simulink model "basic_IO_qarm_mini"  (R2024a)
settings: Solver=ode1  StartTime=0.0  StopTime=inf  FixedStep=1/30  RelTol=1e-3  EnableMultiTasking=on
undefined symbols (not defined in the file): gcbh, HIL, JPEG, qc_get_step_size, video_display_show
libraries: quarc_library x11, simulink x1
settings Model: Creator=msaravanan  LastModifiedBy=Edu-Sivamani
settings SolverCC: PositivePriorityOrder=on
settings HardwareCC: ProdBitPerLong=64  ProdLargestAtomicInteger=LongLong  ProdLargestAtomicFloat=Double  ProdLongLongMode=on  ProdHWDeviceType=ARM Compatible->ARM 64-bit (LP64)
settings RTWCC: Description=QUARC Linux QBot Platform Target Using Toolchain  SystemTargetFile=quarc_linux_qbot_platform.tlc  Toolchain=QUARC linux_qbot_platform | gmake (64-bit Windows)  BuildConfiguration=Faster Runs
settings STFCustomTargetCC: ConcurrentExecutionCompliant=on  SystemTargetFile=quarc_linux_qbot_platform.tlc
settings GRTTargetCC: ParMdlRefBuildCompliant=off  CompOptLevelCompliant=off  CombineOutputUpdateFcns=off  MatFileLogging=off  CPPClassGenCompliant=off  GRTInterface=on  ExtMode=on  ExtModeMexFile=quarc_comm  ExtModeMexArgs='-w -d /tmp -uri %u','tcpip://192.168.2.101:17002'

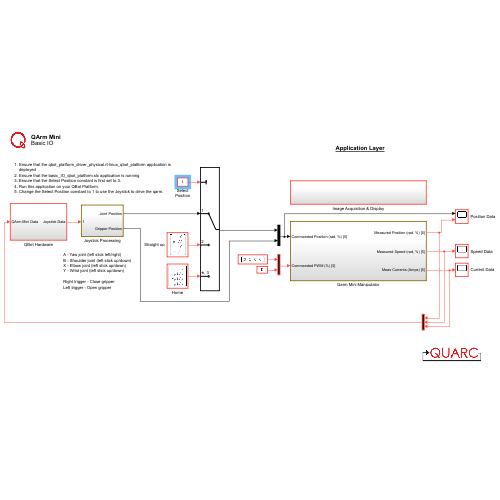
[thumbnail: Simulink's stored preview of the top-level diagram]
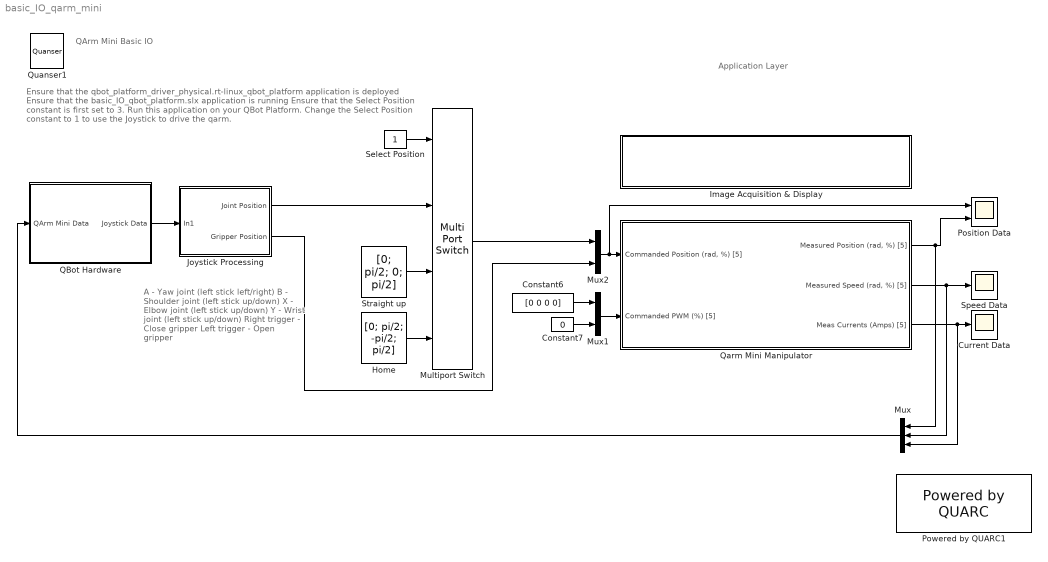
== system basic_IO_qarm_mini ==
  note: A - Yaw joint (left stick left/right)
      | B - Shoulder joint (left stick up/down)
      | X - Elbow joint (left stick up/down)
      | Y - Wrist joint (left stick up/down)
      |
      | Right trigger - Close gripper
      | Left trigger - Open gripper
  note: Ensure that the qbot_platform_driver_physical.rt-linux_qbot_platform application is deployed
      | Ensure that the basic_IO_qbot_platform.slx application is running
      | Ensure that the Select Position constant is first set to 3.
      | Run this application on your QBot Platform.
      | Change the Select Position constant to 1 to use the Joystick to drive the qarm.
  note: QArm Mini
      | Basic IO
  note: Application Layer
  Constant6 : Constant  Value=[0 0 0 0]  SampleTime=qc_get_step_size
  Constant7 : Constant  Value=0  SampleTime=qc_get_step_size
  Current Data : Scope
  Home : Constant  Value=[0; pi/2; -pi/2; pi/2]  VectorParams1D=off  SampleTime=qc_get_step_size
  Image Acquisition & Display : Subsystem
  Joystick Processing : Subsystem
  Multiport Switch : MultiPortSwitch  SaturateOnIntegerOverflow=off  InputSameDT=off
  Mux : Mux  Inputs=3
  Mux1 : Mux  Inputs=2
  Mux2 : Mux  Inputs=2
  Position Data : Scope  NumInputPorts=2
  Powered by QUARC1 : quarc_library/Logos/Powered by QUARC
  QBot Hardware : Subsystem
  Qarm Mini Manipulator : Subsystem
  Quanser1 : quarc_library/Logos/Quanser
  Select Position : Constant  SampleTime=qc_get_step_size
  Speed Data : Scope
  Straight up : Constant  Value=[0; pi/2; 0; pi/2]  VectorParams1D=off  SampleTime=qc_get_step_size
  wires:
  Mux2/1 -> Position Data/1, Qarm Mini Manipulator/1("Commanded Position (rad, %) [5]")
  Constant7/1 -> Mux1/2
  Joystick Processing/2(Gripper Position) -> Mux2/2
  Mux1/1 -> Qarm Mini Manipulator/2(Commanded PWM (%) [5])
  Constant6/1 -> Mux1/1
  Multiport Switch/1 -> Mux2/1
  Qarm Mini Manipulator/1("Measured Position (rad, %) [5]") -> Mux/1, Position Data/2
  Qarm Mini Manipulator/3(Meas Currents (Amps) [5]) -> Mux/3, Current Data/1
  Qarm Mini Manipulator/2("Measured Speed (rad, %) [5]") -> Mux/2, Speed Data/1
  Straight up/1 -> Multiport Switch/3
  QBot Hardware/1(Joystick Data) -> Joystick Processing/1(In1)
  Select Position/1 -> Multiport Switch/1
  Home/1 -> Multiport Switch/4
  Joystick Processing/1(Joint Position) -> Multiport Switch/2
  Mux/1 -> QBot Hardware/1(QArm Mini Data)

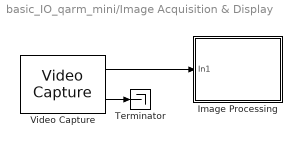
== system basic_IO_qarm_mini/Image Acquisition & Display ==
  Image Processing : Subsystem  LoadFcn=set_param(gcbh, 'UserData', gcb);  StartFcn=video_display_show([gcb, '/Video Display'], 'add', gcb);  mask(Video Compressed Display){algorithm=JPEG, quality=50, sample_time=-1, use_hardware=on}
      mask prompts: algorithm "Compression algorithm:"; quality "Compression quality (0-100):"; sample_time "Sample time (seconds):"; use_hardware "Use hardware acceleration for video display"
      mask help: Displays a video stream on the host, using compression to minimize bandwidth.
      mask init:
      | qc_set_display('Video\nCompressed\nDisplay');
      settings: UndoDeleteFcn=set_param(gcbh, 'UserData', gcb);  OpenFcn=video_display_show([gcb, '/Video Display'], 'show', gcb);  PreDeleteFcn=video_display_show([gcb, '/Video Display'], 'delete');
      settings: CopyFcn=|
      | set_param(gcbh, 'UserData', gcb);
      | set_param(gcbh, 'LinkStatus', 'none');
      settings: NameChangeFcn=|
      | video_display_show([get_param(gcbh, 'UserData'), '/Video Display'], 'rename', [gcb, '/Video Display']);
      | video_display_show([gcb, '/Video Display'], 'add', gcb);
      | set_param(gcbh, 'UserData', gcb);
      mask Help: web(qc_get_block_help_path(gcb));
      mask TypeOptions algorithm: Image Compress/algorithm
      mask TypeOptions quality: Image Compress/quality
      mask TypeOptions sample_time: Video Display/sample_time
      mask TypeOptions use_hardware: Video Display/use_hardware
      mask Display:
      | patch([0.98591 0.98591 0.62618 0.59072 0.56147   0.536   0.536  0.5441 0.56912 0.59207 0.60881 0.62276 0.63527 0.64364  0.6485  0.6485 0.64706 0.64499 0.63662 0.62411 0.61232 0.59837 0.58307 0.56147   0.536   0.536  0.5441  0.5747 0.60953 0.63662 0.67001  0.7034 0.72851 0.75425 0.77927 0.80294 0.82454 0.84119 0.85865 0.87395 0.88574 0.89339  0.8969 0.89969 0.89969 0.89267  0.8816 0.87044 0.85649  0.8384 0.81824 0.80294 0.78764 0.77513 0.76676 0.75776 0.76397 0.77513 0.79178 0.80987 0.82796 0.84326 0.86207 0.98528],[0.18689 0.05522 0.05522 0.05171 0.05171    0.05 0.18338 0.18338 0.19148 0.20435 0.22298 0.24863 0.28589 0.33125 0.38138 0.55139 0.59801 0.63761 0.68189 0.72149 0.74939 0.76694 0.77855 0.79367 0.79952 0.92768 0.92768 0.92768 0.92417 0.92066 0.91364  0.9032 0.89384 0.88106 0.86594 0.85073 0.82634 0.80537 0.77855 0.74363 0.70403 0.65858 0.61079 0.59099 0.41513 0.37202 0.31847 0.29048 0.25556 0.23342  0.2102 0.19382 0.18221 0.17285 0.16943 0.16124  0.1589 0.16241 0.16709 0.17168  0.1787 0.18221 0.18689 0.18689],[0.9,0.90,0.91])
      | patch([0.536 0.52601 0.46823 0.44528 0.41603 0.39101 0.35555 0.33116 0.31451 0.29291  0.2804 0.26717 0.25322 0.23999 0.22406 0.20732 0.19337 0.17528 0.15935 0.14396 0.13217 0.11759 0.10922 0.10085 0.09671 0.09392 0.09041 0.08906 0.08906 0.09464  0.0995 0.10778 0.11894 0.13145 0.14675 0.16349 0.17672 0.19409 0.20732 0.22406 0.23999 0.26159 0.27833 0.29849 0.31793 0.33602 0.35411 0.37085 0.39245 0.41603   0.536   0.536 0.53159 0.46409   0.446 0.42026 0.39587 0.37571 0.36113 0.34925 0.34088 0.33809 0.33809 0.34088 0.34583 0.35627 0.36392 0.38129 0.39587 0.41117 0.42719 0.44672  0.4676 0.48353 0.48353 0.52394   0.536],[0.05 0.04829 0.04712 0.04712 0.04829 0.05063 0.05405 0.05873 0.06107 0.06692 0.07043 0.07619 0.08087 0.08672 0.09482 0.10652 0.11696 0.13325  0.1508 0.17168 0.19499 0.22415 0.25439 0.28472 0.31379 0.35456 0.38489 0.41513 0.58055 0.63878 0.68774 0.72149 0.75641 0.78089 0.80537 0.82859 0.84029 0.85658 0.86594 0.87404  0.8834 0.89267 0.90086 0.90788 0.91247 0.91832 0.92066   0.923 0.92651 0.92768 0.92768 0.79952 0.79952 0.79952 0.79718 0.78899 0.77153 0.75056 0.72149 0.68072 0.62249  0.5549 0.41396 0.37085 0.33242 0.28121 0.25205 0.22181 0.20552 0.19499 0.18572 0.18221 0.17753 0.17636 0.17753  0.1787  0.1787],[0.9,0.90,0.91])
      | disp('Video\nCompressed\nDisplay');
  Terminator : Terminator
  Video Capture : quarc_library/Multimedia/Video Capture  source=device  device=7  filename=sample_movie.mov  value=[0 0; 0 0]  resolution=640 x 360  width=640  height=360  output_format=MATLAB RGB (HxWx3)  data_type=uint8  sample_time=qc_get_step_size * ceil(1 / 60.0 / qc_get_step_size)  brightness_override=Do not override  brightness=50.0  contrast_override=Do not override  contrast=50.0  hue_override=Do not override  hue=50.0  saturation_override=Do not override  saturation=50.0  sharpness_override=Do not override  sharpness=50.0  gamma_override=Do not override  gamma=50.0  coloreffect_override=Do not override  coloreffect=None  whitebalance_override=Do not override  whitebalance=50.0  backlightcompensation_override=Do not override  backlightcompensation=0.0  gain_override=Do not override  gain=50.0  pan_override=Do not override  pan=50.0  tilt_override=Do not override  tilt=50.0  roll_override=Do not override  roll=50.0  zoom_override=Do not override  zoom=0.0  exposure_override=Do not override  exposure=50.0  iris_override=Do not override  iris=50.0  mirror_override=Do not override  mirror=None  focus_override=Do not override  focus=0.0
      settings: SourceProductName=QUARC Targets
  wires:
  Video Capture/1 -> Image Processing/1(In1)
  Video Capture/2 -> Terminator/1

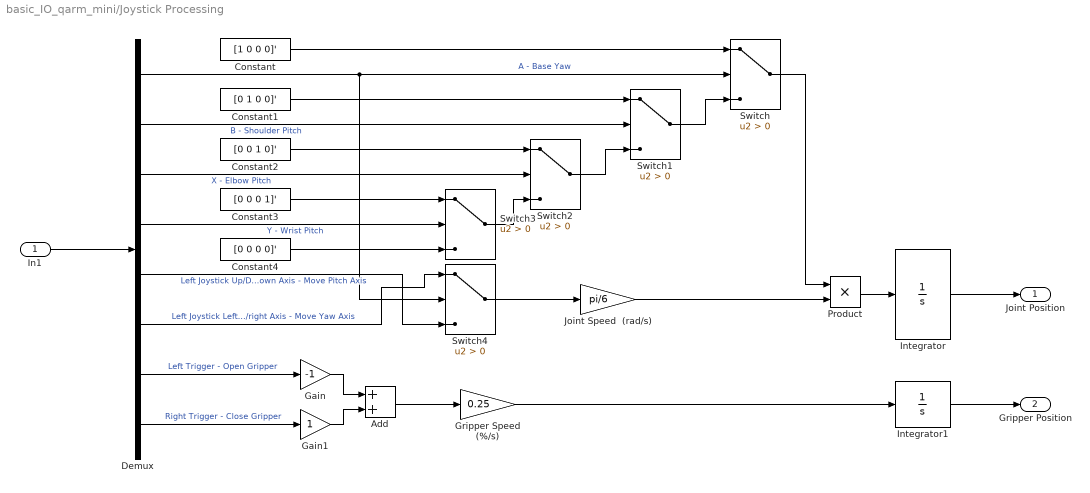
== system basic_IO_qarm_mini/Joystick Processing ==
  In1 : Inport
  Add : Sum
  Constant : Constant  Value=[1 0 0 0]'
  Constant1 : Constant  Value=[0 1 0 0]'
  Constant2 : Constant  Value=[0 0 1 0]'
  Constant3 : Constant  Value=[0 0 0 1]'
  Constant4 : Constant  Value=[0 0 0 0]'
  Demux : Demux  Outputs=8
  Gain : Gain  Gain=-1
  Gain1 : Gain
  Gripper Speed (%/s) : Gain  Gain=0.25
  Integrator : Integrator  InitialCondition=[0; pi/2; -pi/2; pi/2]  LimitOutput=on  UpperSaturationLimit=[5*pi/4, pi, 0, 3*pi/4]'  LowerSaturationLimit=[-pi/2. 0, -3*pi/4, 0]'
  Integrator1 : Integrator  InitialCondition=0.5  LimitOutput=on  UpperSaturationLimit=1  LowerSaturationLimit=0
  Joint Speed  (rad/s) : Gain  Gain=pi/6
  Product : Product
  Switch{,1..4} (5 alike) : Switch  Criteria=u2 > Threshold  SaturateOnIntegerOverflow=off  InputSameDT=off
  Joint Position : Outport
  Gripper Position : Outport  Port=2
  wires:
  In1/1 -> Demux/1
  Demux/1 -> Switch4/2, Switch/2  "A - Base Yaw"
  Constant/1 -> Switch/1
  Switch1/1 -> Switch/3
  Demux/2 -> Switch1/2  "B - Shoulder Pitch"
  Constant1/1 -> Switch1/1
  Demux/3 -> Switch2/2  "X - Elbow Pitch"
  Demux/4 -> Switch3/2  "Y - Wrist Pitch"
  Constant2/1 -> Switch2/1
  Constant3/1 -> Switch3/1
  Constant4/1 -> Switch3/3
  Demux/5 -> Switch4/3  "Left Joystick Up/Down Axis - Move Pitch Axis"
  Demux/6 -> Switch4/1  "Left Joystick Left/right Axis - Move Yaw Axis"
  Switch2/1 -> Switch1/3
  Switch3/1 -> Switch2/3
  Switch4/1 -> Joint Speed  (rad/s)/1
  Switch/1 -> Product/1
  Joint Speed  (rad/s)/1 -> Product/2
  Product/1 -> Integrator/1
  Integrator/1 -> Joint Position/1
  Demux/7 -> Gain/1  "Left Trigger - Open Gripper"
  Demux/8 -> Gain1/1  "Right Trigger - Close Gripper"
  Gain/1 -> Add/1
  Gain1/1 -> Add/2
  Add/1 -> Gripper Speed (%/s)/1
  Gripper Speed (%/s)/1 -> Integrator1/1
  Integrator1/1 -> Gripper Position/1

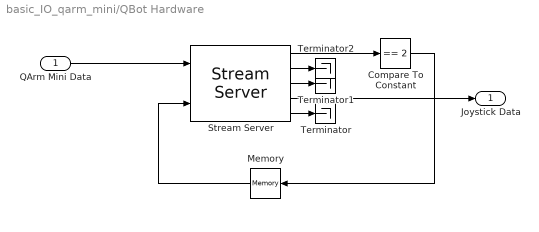
== system basic_IO_qarm_mini/QBot Hardware ==
  QArm Mini Data : Inport
  Compare To Constant : simulink/Logic and Bit Operations/Compare To Constant  relop===  const=2  OutDataTypeStr=boolean
  Memory : Memory  InheritSampleTime=on
  Stream Server : quarc_library/Communications/Basic/Stream Server  uri_source=Specify via dialog (do not evaluate)  uri=tcpip://localhost:18889  send_buffer_size=15*8  receive_buffer_size=8*8  byte_order=little endian (Intel - LSB first)  optimization=Minimum latency  send_options=Send most recent data  receive_options=Receive most recent data  default_value=zeros(1,8)  sample_time=qc_get_step_size  active=on  implementation=Use blocking I/O in a separate thread  send_fifo_size=1000  receive_fifo_size=1000  send_priority=0  receive_priority=0  send_dimensions=off  receive_dimensions=off  max_dimensions=-1  data_type=Inherited via back propagation  type_expr=BusObject
      settings: AttributesFormatString="\"tcpip://localhost:18889\""
  Terminator : Terminator
  Terminator1 : Terminator
  Terminator2 : Terminator
  Joystick Data : Outport
  wires:
  Stream Server/1 -> Compare To Constant/1
  QArm Mini Data/1 -> Stream Server/1
  Compare To Constant/1 -> Memory/1
  Memory/1 -> Stream Server/2
  Stream Server/4 -> Joystick Data/1
  Stream Server/5 -> Terminator/1
  Stream Server/3 -> Terminator1/1
  Stream Server/2 -> Terminator2/1

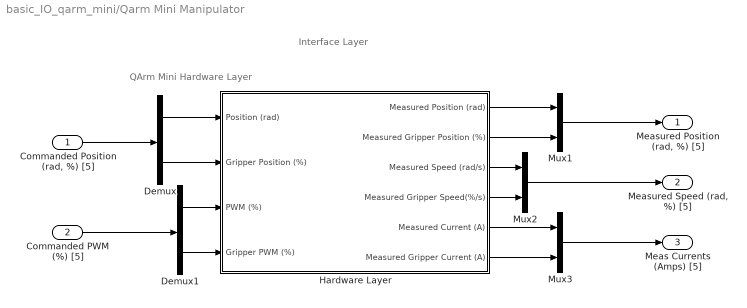
== system basic_IO_qarm_mini/Qarm Mini Manipulator ==
  note: Interface Layer
  note: QArm Mini Hardware Layer
  "Commanded Position (rad, %) [5]" : Inport
  Commanded PWM (%) [5] : Inport  Port=2
  Demux : Demux  Outputs=[4 1]
  Demux1 : Demux  Outputs=[4 1]
  Hardware Layer : Subsystem
  Mux1 : Mux  Inputs=2
  Mux2 : Mux  Inputs=2
  Mux3 : Mux  Inputs=2
  "Measured Position (rad, %) [5]" : Outport
  "Measured Speed (rad, %) [5]" : Outport  Port=2
  Meas Currents (Amps) [5] : Outport  Port=3
  wires:
  Demux/2 -> Hardware Layer/2(Gripper Position (%))
  Hardware Layer/1(Measured Position (rad)) -> Mux1/1
  Demux1/2 -> Hardware Layer/4(Gripper PWM (%))
  Hardware Layer/2(Measured Gripper Position (%)) -> Mux1/2
  Hardware Layer/3(Measured Speed (rad/s)) -> Mux2/1
  Hardware Layer/4(Measured Gripper Speed(%/s)) -> Mux2/2
  Hardware Layer/5(Measured Current (A)) -> Mux3/1
  Hardware Layer/6(Measured Gripper Current (A)) -> Mux3/2
  Mux3/1 -> Meas Currents (Amps) [5]/1
  Mux2/1 -> "Measured Speed (rad, %) [5]"/1
  Mux1/1 -> "Measured Position (rad, %) [5]"/1
  "Commanded Position (rad, %) [5]"/1 -> Demux/1
  Demux/1 -> Hardware Layer/1(Position (rad))
  Demux1/1 -> Hardware Layer/3(PWM (%))
  Commanded PWM (%) [5]/1 -> Demux1/1

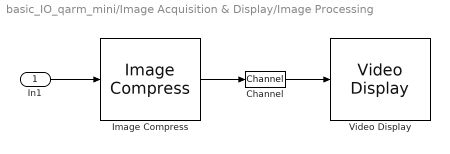
== system basic_IO_qarm_mini/Image Acquisition & Display/Image Processing ==
  In1 : Inport
  Channel : quarc_library/Signal Routing/Channel  channel=0  buffer_size=1
  Image Compress : quarc_library/Image Processing/Generic/Image Compress  algorithm=JPEG  source=Internal dialog parameter  quality=quality  output_dim=-1
  Video Display : quarc_library/Multimedia/Video Display  Tag=basic_IO_qarm_mini/Image Acquisition & Display/Image Processing/Video Display  sample_time=sample_time  use_hardware=on
  wires:
  Image Compress/1 -> Channel/1
  In1/1 -> Image Compress/1
  Channel/1 -> Video Display/1

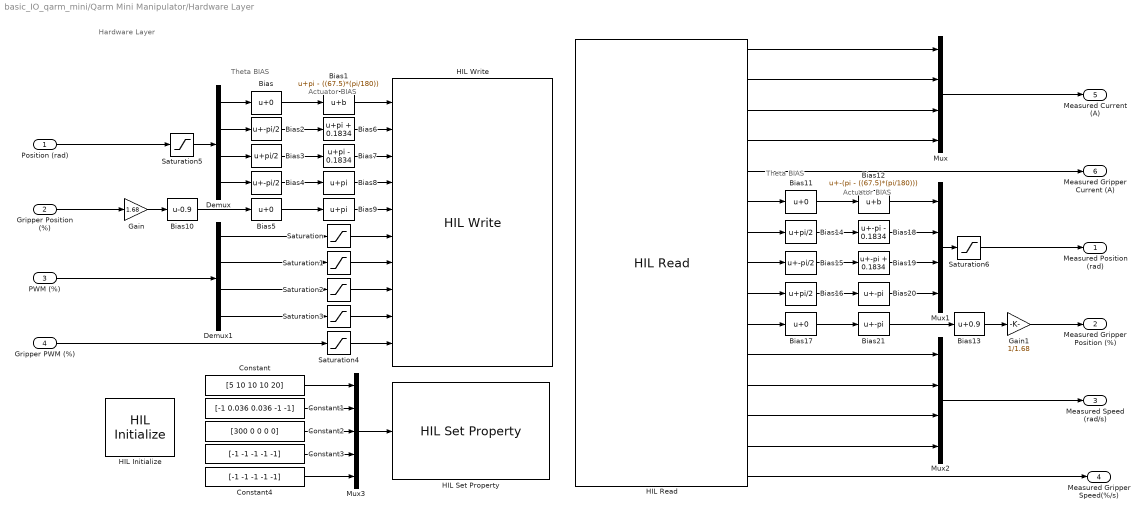
== system basic_IO_qarm_mini/Qarm Mini Manipulator/Hardware Layer ==
  note: Hardware Layer
  note: Actuator BIAS
  note: Theta BIAS
  note: Actuator BIAS
  note: Theta BIAS
  Position (rad) : Inport
  Gripper Position (%) : Inport  Port=2
  PWM (%) : Inport  Port=3
  Gripper PWM (%) : Inport  Port=4
  Bias{,5,11,17} (4 alike) : Bias  SaturateOnIntegerOverflow=off
  Bias1 : Bias  Bias=pi - ((67.5)*(pi/180))  SaturateOnIntegerOverflow=off
  Bias10 : Bias  Bias=-0.9  SaturateOnIntegerOverflow=off
  Bias12 : Bias  Bias=-(pi - ((67.5)*(pi/180)))  SaturateOnIntegerOverflow=off
  Bias13 : Bias  Bias=0.9  SaturateOnIntegerOverflow=off
  Bias14 : Bias  Bias=pi/2  SaturateOnIntegerOverflow=off
  Bias15 : Bias  Bias=-pi/2  SaturateOnIntegerOverflow=off
  Bias16 : Bias  Bias=pi/2  SaturateOnIntegerOverflow=off
  Bias18 : Bias  Bias="-pi -  0.1834"  SaturateOnIntegerOverflow=off
  Bias19 : Bias  Bias="-pi +  0.1834"  SaturateOnIntegerOverflow=off
  Bias2 : Bias  Bias=-pi/2  SaturateOnIntegerOverflow=off
  Bias20 : Bias  Bias=-pi  SaturateOnIntegerOverflow=off
  Bias21 : Bias  Bias=-pi  SaturateOnIntegerOverflow=off
  Bias3 : Bias  Bias=pi/2  SaturateOnIntegerOverflow=off
  Bias4 : Bias  Bias=-pi/2  SaturateOnIntegerOverflow=off
  Bias6 : Bias  Bias=pi + 0.1834  SaturateOnIntegerOverflow=off
  Bias7 : Bias  Bias="pi -  0.1834"  SaturateOnIntegerOverflow=off
  Bias8 : Bias  Bias=pi  SaturateOnIntegerOverflow=off
  Bias9 : Bias  Bias=pi  SaturateOnIntegerOverflow=off
  Constant : Constant  Value=[5 10 10 10 20]
  Constant1 : Constant  Value=[-1 0.036 0.036 -1 -1]
  Constant2 : Constant  Value=[300 0 0 0 0]
  Constant3 : Constant  Value=[-1 -1 -1 -1 -1]
  Constant4 : Constant  Value=[-1 -1 -1 -1 -1]
  Demux : Demux
  Demux1 : Demux
  Gain : Gain  Gain=1.68
  Gain1 : Gain  Gain=1/1.68
  HIL Initialize : quarc_library/Data Acquisition/Generic/Configuration/HIL Initialize  object_name=HIL-1  board_type=qarm_mini  board_number=0  board_options=j0_mode=0;j1_mode=0;j2_mode=0;j3_mode=0;gripper_mode=0;j0_profile_velocity=6.2832;j0_profile_acceleration=6.2832;j1_profile_velocity=6.2832;j1_profile_acceleration=6.2832;j2_profile_velocity=6.2832;j2_profile_acceleration=6.2832;j3_profile_velocity=6.2832;j3_profile_acceleration=6.2832;gripper_profile_velocity=6.2832;gripper_profile_acceleration=6.2832;  exclusive=off  active=on  hardware_clocks=[]  clock_modes=[]  initial_clock_frequencies=[]  set_clock_params_at_start=off  set_clock_params_at_switch_in=off  set_clock_frequencies_at_start=off  set_clock_frequencies_at_switch_in=off  analog_input_channels=[0:4]  analog_input_configurations=[]  analog_input_maximums=[100 3.21 3.21 3.21 100]  analog_input_minimums=[-100 -3.21 -3.21 -3.21 -100]  set_analog_input_params_at_start=off  set_analog_input_params_at_switch_in=off  analog_output_channels=[]  analog_output_maximums=[]  analog_output_minimums=[]  initial_analog_outputs=[]  final_analog_outputs=[]  watchdog_analog_outputs=[]  set_analog_output_params_at_start=off  set_analog_output_params_at_switch_in=off  set_analog_outputs_at_start=off  set_analog_outputs_at_switch_in=off  set_analog_outputs_at_terminate=off  set_analog_outputs_at_switch_out=off  set_analog_outputs_on_watchdog=off  digital_input_channels=[]  digital_output_channels=[]  digital_output_configuration=[]  initial_digital_outputs=[]  final_digital_outputs=[]  watchdog_digital_outputs=[]  set_digital_output_params_at_start=off  set_digital_output_params_at_switch_in=off  set_digital_outputs_at_start=off  set_digital_outputs_at_switch_in=off  set_digital_outputs_at_terminate=off  set_digital_outputs_at_switch_out=off  set_digital_outputs_on_watchdog=off  encoder_channels=[]  quadrature=[]  encoder_filter_frequency=[]  initial_encoder_counts=[]  set_encoder_params_at_start=off  set_encoder_params_at_switch_in=off  set_encoder_counts_at_start=off  set_encoder_counts_at_switch_in=off  pwm_channels=[]  pwm_modes=[]  pwm_frequency=[]  pwm_configuration=[]  pwm_alignment=[]  pwm_polarity=[]  pwm_leading_deadband=[]  pwm_trailing_deadband=[]  initial_pwm_outputs=[]  final_pwm_outputs=[]  watchdog_pwm_outputs=[]  set_pwm_params_at_start=off  set_pwm_params_at_switch_in=off  set_pwm_outputs_at_start=off  set_pwm_outputs_at_switch_in=off  set_pwm_outputs_at_terminate=off  set_pwm_outputs_at_switch_out=off  set_pwm_outputs_on_watchdog=off  other_output_channels=[]  initial_other_outputs=[]  final_other_outputs=[]  watchdog_other_outputs=[]  set_other_outputs_at_start=off  set_other_outputs_at_switch_in=off  set_other_outputs_at_terminate=off  set_other_outputs_at_switch_out=off  set_other_outputs_on_watchdog=off
  HIL Read : quarc_library/Data Acquisition/Generic/Immediate I//O/HIL Read  object_name=HIL-1  analog_channels=[0:4]  encoder_channels=[]  digital_channels=[]  other_channels=[1000:1004 3000:3004]  sample_time=qc_get_step_size  active=on  vector_output=off  data_type_mode=Inherit via back propagation  encoder_data_type=double  digital_data_type=boolean
  HIL Set Property : quarc_library/Data Acquisition/Generic/Configuration/HIL Set Property  object_name=HIL-1  property_type=2  property_codes=[128:152]  property_source=2  property_value_num=0  set_at_start=on  sample_time=-1  active=off
      settings: AttributesFormatString=(%<object_name>)  SourceProductName=QUARC Targets
  HIL Write : quarc_library/Data Acquisition/Generic/Immediate I//O/HIL Write  object_name=HIL-1  analog_channels=[]  pwm_channels=[]  digital_channels=[]  other_channels=[1000:1004 11000:11004]  sample_time=qc_get_step_size  active=on  vector_input=off
  Mux : Mux
  Mux1 : Mux
  Mux2 : Mux
  Mux3 : Mux  Inputs=5
  Saturation{,1..4} (5 alike) : Saturate
  Saturation5 : Saturate  UpperLimit=[5*pi/4, pi, 0, 3*pi/4]'  LowerLimit=[-pi/2. 0, -3*pi/4, 0]'
  Saturation6 : Saturate  UpperLimit=[5*pi/4, pi, 0, 3*pi/4]'  LowerLimit=[-pi/2. 0, -3*pi/4, 0]'
  Measured Position (rad) : Outport
  Measured Gripper Position (%) : Outport  Port=2
  Measured Speed (rad/s) : Outport  Port=3
  Measured Gripper Speed(%/s) : Outport  Port=4
  Measured Current (A) : Outport  Port=5
  Measured Gripper Current (A) : Outport  Port=6
  wires:
  Position (rad)/1 -> Saturation5/1
  Demux/2 -> Bias2/1
  Demux/3 -> Bias3/1
  Demux/4 -> Bias4/1
  Bias/1 -> Bias1/1
  Bias1/1 -> HIL Write/1
  Bias2/1 -> Bias6/1
  Bias6/1 -> HIL Write/2
  Bias3/1 -> Bias7/1
  Bias7/1 -> HIL Write/3
  Bias4/1 -> Bias8/1
  Bias8/1 -> HIL Write/4
  Bias5/1 -> Bias9/1
  Bias9/1 -> HIL Write/5
  Gain/1 -> Bias10/1
  PWM (%)/1 -> Demux1/1
  Gripper PWM (%)/1 -> Saturation4/1
  Saturation/1 -> HIL Write/6
  Saturation1/1 -> HIL Write/7
  Saturation2/1 -> HIL Write/8
  Saturation3/1 -> HIL Write/9
  Saturation4/1 -> HIL Write/10
  HIL Read/1 -> Mux/1
  HIL Read/2 -> Mux/2
  HIL Read/3 -> Mux/3
  HIL Read/4 -> Mux/4
  Mux/1 -> Measured Current (A)/1
  HIL Read/5 -> Measured Gripper Current (A)/1
  Bias14/1 -> Bias18/1
  Bias15/1 -> Bias19/1
  Bias17/1 -> Bias21/1
  Bias11/1 -> Bias12/1
  Bias16/1 -> Bias20/1
  HIL Read/6 -> Bias11/1
  HIL Read/7 -> Bias14/1
  HIL Read/8 -> Bias15/1
  HIL Read/9 -> Bias16/1
  HIL Read/10 -> Bias17/1
  Bias21/1 -> Bias13/1
  Bias13/1 -> Gain1/1
  Gain1/1 -> Measured Gripper Position (%)/1
  Mux1/1 -> Saturation6/1
  HIL Read/11 -> Mux2/1
  HIL Read/12 -> Mux2/2
  HIL Read/13 -> Mux2/3
  HIL Read/14 -> Mux2/4
  Mux2/1 -> Measured Speed (rad/s)/1
  HIL Read/15 -> Measured Gripper Speed(%/s)/1
  Constant/1 -> Mux3/1
  Constant1/1 -> Mux3/2
  Constant2/1 -> Mux3/3
  Constant3/1 -> Mux3/4
  Constant4/1 -> Mux3/5
  Mux3/1 -> HIL Set Property/1
  Bias12/1 -> Mux1/1
  Bias18/1 -> Mux1/2
  Bias19/1 -> Mux1/3
  Bias20/1 -> Mux1/4
  Demux1/1 -> Saturation/1
  Demux1/2 -> Saturation1/1
  Demux1/3 -> Saturation2/1
  Demux1/4 -> Saturation3/1
  Demux/1 -> Bias/1
  Saturation5/1 -> Demux/1
  Saturation6/1 -> Measured Position (rad)/1
  Gripper Position (%)/1 -> Gain/1
  Bias10/1 -> Bias5/1
